simulink model "ParrotMinidroneKeyboardControl"  (R2025b)
settings: Solver=ode3  StartTime=0  StopTime=TFinal  FixedStep=Ts  RelTol=1e-3  EnableMultiTasking=on
values from neighbouring files (symbols this model uses):
  sensorCalibrationData = [0.09 -0.06 -9.473 -0.0095 -0.0075 0.0015 101270.95 0.2]    [sensorCalibration.mat]
undefined symbols (not defined in the file or in its folder): Command, ft, gcbh, init, m, Rec, s, SDTV, Sensors, States, stop_time, takeOffDuration, Ts, Vehicle, vrmfunc, VTs
libraries: simulink x16, aerolibconvert2 x4, SignalEditorBlockLib x2, environmentLibrary x2, visionconversions x2, visiongeotforms x2, aerolibutil x2, aerolibanimutils x1, aerolibnav x1, vrlib x1
(part 2 of 2)

== system ParrotMinidroneKeyboardControl/Simulink 3D Visualization/Simulink 3D/Euler to VR/Axis Angle Vector ==
  e0 : Inport
  2 : Gain  Gain=2  SaturateOnIntegerOverflow=on  OutDataTypeStr=Inherit: Same as input  ParamDataTypeStr=Inherit: Same as input
  Constant : Constant  Value=1e-6
  Demux : Demux  Outputs=[1 3 ]
      settings: DisplayOption=none
  Mux : Mux  Inputs=2
  Product : Product  Inputs=*/  InputSameDT=on  SaturateOnIntegerOverflow=on  OutDataTypeStr=Inherit: Same as first input
  Switch : Switch  Criteria=u2 ~= 0  SaturateOnIntegerOverflow=off  InputSameDT=off
  Trigonometric Function : Trigonometry
  Trigonometric Function2 : Trigonometry  Operator=acos
  e0_norm : Outport  VectorParamsAs1DForOutWhenUnconnected=off
  wires:
  Demux/1 -> Trigonometric Function2/1
  Demux/2 -> Product/1
  Mux/1 -> e0_norm/1
  Product/1 -> Mux/1
  2/1 -> Mux/2
  Trigonometric Function/1 -> Switch/1, Switch/2
  Trigonometric Function2/1 -> Trigonometric Function/1, 2/1
  e0/1 -> Demux/1
  Constant/1 -> Switch/3
  Switch/1 -> Product/2

== system ParrotMinidroneKeyboardControl/Simulink 3D Visualization/Simulink 3D/Euler to VR/Quaternion Normalization ==
  e0 : Inport
  1/2 : Gain  Gain=1/2  SaturateOnIntegerOverflow=on  OutDataTypeStr=Inherit: Same as input  ParamDataTypeStr=Inherit: Same as input
  Demux : Demux  Outputs=[1 3]
      settings: DisplayOption=none
  Mux : Mux  Inputs=2
  Product : Product  InputSameDT=on  SaturateOnIntegerOverflow=on  OutDataTypeStr=Inherit: Same as first input
  Trigonometric Function : Trigonometry
  Trigonometric Function1 : Trigonometry  Operator=cos
  e0_norm : Outport  VectorParamsAs1DForOutWhenUnconnected=off
  wires:
  Trigonometric Function1/1 -> Mux/1
  Demux/2 -> Product/2
  Demux/1 -> 1/2/1
  Mux/1 -> e0_norm/1
  Product/1 -> Mux/2
  Trigonometric Function/1 -> Product/1
  1/2/1 -> Trigonometric Function1/1, Trigonometric Function/1
  e0/1 -> Demux/1

== system ParrotMinidroneKeyboardControl/Simulink 3D Visualization/Simulink 3D/Euler to VR/Quaternion Normalization1 ==
  e0 : Inport
  1/2 : Gain  Gain=1/2  SaturateOnIntegerOverflow=on  OutDataTypeStr=Inherit: Same as input  ParamDataTypeStr=Inherit: Same as input
  Demux : Demux  Outputs=[1 3]
      settings: DisplayOption=none
  Mux : Mux  Inputs=2
  Product : Product  InputSameDT=on  SaturateOnIntegerOverflow=on  OutDataTypeStr=Inherit: Same as first input
  Trigonometric Function : Trigonometry
  Trigonometric Function1 : Trigonometry  Operator=cos
  e0_norm : Outport  VectorParamsAs1DForOutWhenUnconnected=off
  wires:
  e0/1 -> Demux/1
  1/2/1 -> Trigonometric Function/1, Trigonometric Function1/1
  Trigonometric Function/1 -> Product/1
  Product/1 -> Mux/2
  Mux/1 -> e0_norm/1
  Demux/1 -> 1/2/1
  Demux/2 -> Product/2
  Trigonometric Function1/1 -> Mux/1

== system ParrotMinidroneKeyboardControl/Simulink 3D Visualization/Simulink 3D/Euler to VR/Quaternion Normalization2 ==
  e0 : Inport
  1/2 : Gain  Gain=1/2  SaturateOnIntegerOverflow=on  OutDataTypeStr=Inherit: Same as input  ParamDataTypeStr=Inherit: Same as input
  Demux : Demux  Outputs=[1 3]
      settings: DisplayOption=none
  Mux : Mux  Inputs=2
  Product : Product  InputSameDT=on  SaturateOnIntegerOverflow=on  OutDataTypeStr=Inherit: Same as first input
  Trigonometric Function : Trigonometry
  Trigonometric Function1 : Trigonometry  Operator=cos
  e0_norm : Outport  VectorParamsAs1DForOutWhenUnconnected=off
  wires:
  Trigonometric Function1/1 -> Mux/1
  Demux/2 -> Product/2
  Demux/1 -> 1/2/1
  Mux/1 -> e0_norm/1
  Product/1 -> Mux/2
  Trigonometric Function/1 -> Product/1
  1/2/1 -> Trigonometric Function1/1, Trigonometric Function/1
  e0/1 -> Demux/1

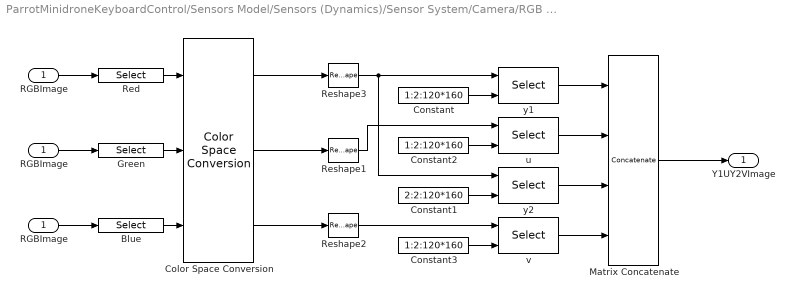
== system ParrotMinidroneKeyboardControl/Sensors Model/Sensors (Dynamics)/Sensor System/Camera/RGB to Y1UY2V1 ==
  RGBImage : Inport  OutDataTypeStr=uint8  PortDimensions=[120 160 3]
  " RGBImage " : InportShadow  OutDataTypeStr=uint8  PortDimensions=[120 160 3]
  Blue : Selector  NumberOfDimensions=3  InputPortWidth=3  IndexOptions=Select all,Select all,Index vector (dialog)  Indices=1,1,3  OutputSizes=1,1,1
  Color Space Conversion : visionconversions/Color Space  Conversion  conversion=Obsolete  conversionActive=R'G'B' to Y'CbCr  wp_str=D65  rec=Rec. 601 (SDTV)  sys=1125/60/2:1  imagePorts=Separate color signals
  Constant : Constant  Value=1:2:120*160
  Constant1 : Constant  Value=2:2:120*160
  Constant2 : Constant  Value=1:2:120*160
  Constant3 : Constant  Value=1:2:120*160
  Green : Selector  NumberOfDimensions=3  InputPortWidth=3  IndexOptions=Select all,Select all,Index vector (dialog)  Indices=1,1,2  OutputSizes=1,1,1
  Matrix Concatenate : Concatenate  NumInputs=4  Mode=Multidimensional array
  "RGBImage " : InportShadow  OutDataTypeStr=uint8  PortDimensions=[120 160 3]
  Red : Selector  NumberOfDimensions=3  InputPortWidth=3  IndexOptions=Select all,Select all,Index vector (dialog)  Indices=1,1,1  OutputSizes=1,1,1
  Reshape1 : Reshape  OutputDimensionality=Customize  OutputDimensions=[1,19200]
  Reshape2 : Reshape  OutputDimensionality=Customize  OutputDimensions=[1,19200]
  Reshape3 : Reshape  OutputDimensionality=Customize  OutputDimensions=[1,19200]
  u : Selector  InputPortWidth=120*160  IndexOptions=Index vector (port)  Indices=[1 3]  OutputSizes=1
  v : Selector  InputPortWidth=120*160  IndexOptions=Index vector (port)  Indices=[1 3]  OutputSizes=1
  y1 : Selector  InputPortWidth=120*160  IndexOptions=Index vector (port)  Indices=[1 3]  OutputSizes=1
  y2 : Selector  InputPortWidth=120*160  IndexOptions=Index vector (port)  Indices=[1 3]  OutputSizes=1
  Y1UY2VImage : Outport  OutDataTypeStr=uint8  PortDimensions=[4 9600]  VectorParamsAs1DForOutWhenUnconnected=off
  wires:
  v/1 -> Matrix Concatenate/4
  y1/1 -> Matrix Concatenate/1
  RGBImage/1 -> Green/1
  Red/1 -> Color Space Conversion/1
  Green/1 -> Color Space Conversion/2
  Blue/1 -> Color Space Conversion/3
  Reshape3/1 -> y1/1, y2/1
  Reshape1/1 -> u/1
  Reshape2/1 -> v/1
  Constant/1 -> y1/2
  Constant1/1 -> y2/2
  Constant2/1 -> u/2
  Constant3/1 -> v/2
  Matrix Concatenate/1 -> Y1UY2VImage/1
  u/1 -> Matrix Concatenate/2
  y2/1 -> Matrix Concatenate/3
  " RGBImage "/1 -> Red/1
  "RGBImage "/1 -> Blue/1
  Color Space Conversion/1 -> Reshape3/1
  Color Space Conversion/2 -> Reshape1/1
  Color Space Conversion/3 -> Reshape2/1

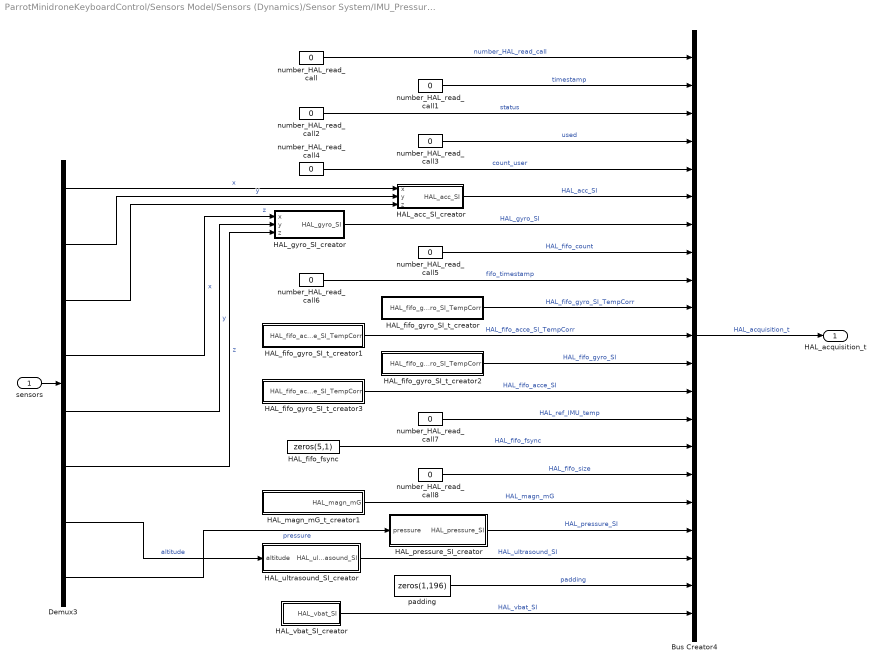
== system ParrotMinidroneKeyboardControl/Sensors Model/Sensors (Dynamics)/Sensor System/IMU_Pressure/HAL_acquisition_creator ==
  sensors : Inport
  Bus Creator4 : BusCreator  Inputs=21  OutDataTypeStr=Bus: HAL_acquisition_t  NonVirtualBus=on
      settings: InheritFromInputs=off
  Demux3 : Demux  Outputs=8
  HAL_acc_SI_creator : Subsystem
  HAL_fifo_fsync : Constant  Value=zeros(5,1)  OutDataTypeStr=uint8
  HAL_fifo_gyro_SI_t_creator : Subsystem
  HAL_fifo_gyro_SI_t_creator1 : Subsystem
  HAL_fifo_gyro_SI_t_creator2 : Subsystem
  HAL_fifo_gyro_SI_t_creator3 : Subsystem
  HAL_gyro_SI_creator : Subsystem
  HAL_magn_mG_t_creator1 : Subsystem
  HAL_pressure_SI_creator : Subsystem
  HAL_ultrasound_SI_creator : Subsystem
  HAL_vbat_SI_creator : Subsystem
  number_HAL_read_call : Constant  Value=0  OutDataTypeStr=int32
  number_HAL_read_call1 : Constant  Value=0  OutDataTypeStr=uint32
  number_HAL_read_call2 : Constant  Value=0  OutDataTypeStr=uint16
  number_HAL_read_call3 : Constant  Value=0  OutDataTypeStr=uint8
  number_HAL_read_call4 : Constant  Value=0  OutDataTypeStr=uint8
  number_HAL_read_call5 : Constant  Value=0  OutDataTypeStr=uint16
  number_HAL_read_call6 : Constant  Value=0  OutDataTypeStr=uint32
  number_HAL_read_call7 : Constant  Value=0  OutDataTypeStr=single
  number_HAL_read_call8 : Constant  Value=0  OutDataTypeStr=int32
  padding : Constant  Value=zeros(1,196)  OutDataTypeStr=uint8
  HAL_acquisition_t : Outport  OutDataTypeStr=Bus: HAL_acquisition_t  VectorParamsAs1DForOutWhenUnconnected=off
  wires:
  HAL_fifo_gyro_SI_t_creator1/1(HAL_fifo_acce_SI_TempCorr) -> Bus Creator4/11  "HAL_fifo_acce_SI_TempCorr"
  HAL_fifo_gyro_SI_t_creator2/1(HAL_fifo_gyro_SI_TempCorr) -> Bus Creator4/12  "HAL_fifo_gyro_SI"
  HAL_fifo_gyro_SI_t_creator3/1(HAL_fifo_acce_SI_TempCorr) -> Bus Creator4/13  "HAL_fifo_acce_SI"
  HAL_magn_mG_t_creator1/1(HAL_magn_mG) -> Bus Creator4/17  "HAL_magn_mG"
  HAL_fifo_fsync/1 -> Bus Creator4/15  "HAL_fifo_fsync"
  HAL_fifo_gyro_SI_t_creator/1(HAL_fifo_gyro_SI_TempCorr) -> Bus Creator4/10  "HAL_fifo_gyro_SI_TempCorr"
  number_HAL_read_call5/1 -> Bus Creator4/8  "HAL_fifo_count"
  number_HAL_read_call8/1 -> Bus Creator4/16  "HAL_fifo_size"
  number_HAL_read_call/1 -> Bus Creator4/1  "number_HAL_read_call"
  number_HAL_read_call2/1 -> Bus Creator4/3  "status"
  number_HAL_read_call3/1 -> Bus Creator4/4  "used"
  number_HAL_read_call6/1 -> Bus Creator4/9  "fifo_timestamp"
  number_HAL_read_call1/1 -> Bus Creator4/2  "timestamp"
  number_HAL_read_call4/1 -> Bus Creator4/5  "count_user"
  padding/1 -> Bus Creator4/20  "padding"
  number_HAL_read_call7/1 -> Bus Creator4/14  "HAL_ref_IMU_temp"
  HAL_vbat_SI_creator/1(HAL_vbat_SI) -> Bus Creator4/21  "HAL_vbat_SI"
  HAL_pressure_SI_creator/1(HAL_pressure_SI) -> Bus Creator4/18  "HAL_pressure_SI"
  Demux3/8 -> HAL_pressure_SI_creator/1(pressure)  "pressure"
  HAL_acc_SI_creator/1(HAL_acc_SI) -> Bus Creator4/6  "HAL_acc_SI"
  Demux3/3 -> HAL_acc_SI_creator/3(z)  "z"
  Demux3/2 -> HAL_acc_SI_creator/2(y)  "y"
  Demux3/1 -> HAL_acc_SI_creator/1(x)  "x"
  HAL_gyro_SI_creator/1(HAL_gyro_SI) -> Bus Creator4/7  "HAL_gyro_SI"
  Demux3/6 -> HAL_gyro_SI_creator/3(z)  "z"
  Demux3/5 -> HAL_gyro_SI_creator/2(y)  "y"
  Demux3/4 -> HAL_gyro_SI_creator/1(x)  "x"
  HAL_ultrasound_SI_creator/1(HAL_ultrasound_SI) -> Bus Creator4/19  "HAL_ultrasound_SI"
  Demux3/7 -> HAL_ultrasound_SI_creator/1(altitude)  "altitude"
  sensors/1 -> Demux3/1
  Bus Creator4/1 -> HAL_acquisition_t/1  "HAL_acquisition_t"

== system ParrotMinidroneKeyboardControl/Sensors Model/Sensors (Feedthrough)/Sensor System/Camera/RGB to Y1UY2V1 ==
  RGBImage : Inport  OutDataTypeStr=uint8  PortDimensions=[120 160 3]
  " RGBImage " : InportShadow  OutDataTypeStr=uint8  PortDimensions=[120 160 3]
  Blue : Selector  NumberOfDimensions=3  InputPortWidth=3  IndexOptions=Select all,Select all,Index vector (dialog)  Indices=1,1,3  OutputSizes=1,1,1
  Color Space Conversion : visionconversions/Color Space  Conversion  conversion=Obsolete  conversionActive=R'G'B' to Y'CbCr  wp_str=D65  rec=Rec. 601 (SDTV)  sys=1125/60/2:1  imagePorts=Separate color signals
  Constant : Constant  Value=1:2:120*160
  Constant1 : Constant  Value=2:2:120*160
  Constant2 : Constant  Value=1:2:120*160
  Constant3 : Constant  Value=1:2:120*160
  Green : Selector  NumberOfDimensions=3  InputPortWidth=3  IndexOptions=Select all,Select all,Index vector (dialog)  Indices=1,1,2  OutputSizes=1,1,1
  Matrix Concatenate : Concatenate  NumInputs=4  Mode=Multidimensional array
  "RGBImage " : InportShadow  OutDataTypeStr=uint8  PortDimensions=[120 160 3]
  Red : Selector  NumberOfDimensions=3  InputPortWidth=3  IndexOptions=Select all,Select all,Index vector (dialog)  Indices=1,1,1  OutputSizes=1,1,1
  Reshape1 : Reshape  OutputDimensionality=Customize  OutputDimensions=[1,19200]
  Reshape2 : Reshape  OutputDimensionality=Customize  OutputDimensions=[1,19200]
  Reshape3 : Reshape  OutputDimensionality=Customize  OutputDimensions=[1,19200]
  u : Selector  InputPortWidth=120*160  IndexOptions=Index vector (port)  Indices=[1 3]  OutputSizes=1
  v : Selector  InputPortWidth=120*160  IndexOptions=Index vector (port)  Indices=[1 3]  OutputSizes=1
  y1 : Selector  InputPortWidth=120*160  IndexOptions=Index vector (port)  Indices=[1 3]  OutputSizes=1
  y2 : Selector  InputPortWidth=120*160  IndexOptions=Index vector (port)  Indices=[1 3]  OutputSizes=1
  Y1UY2VImage : Outport  OutDataTypeStr=uint8  PortDimensions=[4 9600]  VectorParamsAs1DForOutWhenUnconnected=off
  wires:
  v/1 -> Matrix Concatenate/4
  y1/1 -> Matrix Concatenate/1
  RGBImage/1 -> Green/1
  Red/1 -> Color Space Conversion/1
  Green/1 -> Color Space Conversion/2
  Blue/1 -> Color Space Conversion/3
  Reshape3/1 -> y1/1, y2/1
  Reshape1/1 -> u/1
  Reshape2/1 -> v/1
  Constant/1 -> y1/2
  Constant1/1 -> y2/2
  Constant2/1 -> u/2
  Constant3/1 -> v/2
  Matrix Concatenate/1 -> Y1UY2VImage/1
  u/1 -> Matrix Concatenate/2
  y2/1 -> Matrix Concatenate/3
  " RGBImage "/1 -> Red/1
  "RGBImage "/1 -> Blue/1
  Color Space Conversion/1 -> Reshape3/1
  Color Space Conversion/2 -> Reshape1/1
  Color Space Conversion/3 -> Reshape2/1

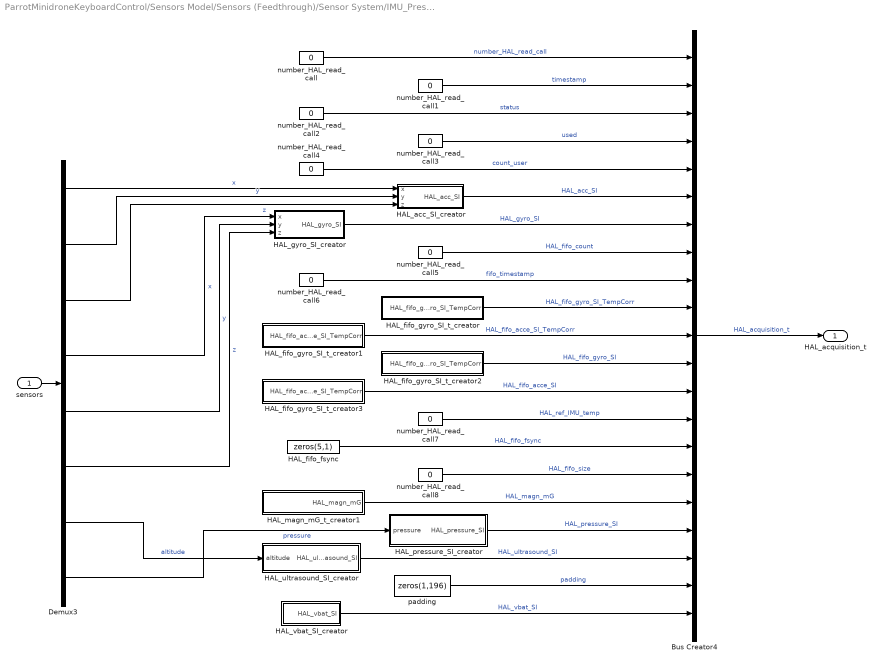
== system ParrotMinidroneKeyboardControl/Sensors Model/Sensors (Feedthrough)/Sensor System/IMU_Pressure/HAL_acquisition_creator ==
  sensors : Inport
  Bus Creator4 : BusCreator  Inputs=21  OutDataTypeStr=Bus: HAL_acquisition_t  NonVirtualBus=on
      settings: InheritFromInputs=off
  Demux3 : Demux  Outputs=8
  HAL_acc_SI_creator : Subsystem
  HAL_fifo_fsync : Constant  Value=zeros(5,1)  OutDataTypeStr=uint8
  HAL_fifo_gyro_SI_t_creator : Subsystem
  HAL_fifo_gyro_SI_t_creator1 : Subsystem
  HAL_fifo_gyro_SI_t_creator2 : Subsystem
  HAL_fifo_gyro_SI_t_creator3 : Subsystem
  HAL_gyro_SI_creator : Subsystem
  HAL_magn_mG_t_creator1 : Subsystem
  HAL_pressure_SI_creator : Subsystem
  HAL_ultrasound_SI_creator : Subsystem
  HAL_vbat_SI_creator : Subsystem
  number_HAL_read_call : Constant  Value=0  OutDataTypeStr=int32
  number_HAL_read_call1 : Constant  Value=0  OutDataTypeStr=uint32
  number_HAL_read_call2 : Constant  Value=0  OutDataTypeStr=uint16
  number_HAL_read_call3 : Constant  Value=0  OutDataTypeStr=uint8
  number_HAL_read_call4 : Constant  Value=0  OutDataTypeStr=uint8
  number_HAL_read_call5 : Constant  Value=0  OutDataTypeStr=uint16
  number_HAL_read_call6 : Constant  Value=0  OutDataTypeStr=uint32
  number_HAL_read_call7 : Constant  Value=0  OutDataTypeStr=single
  number_HAL_read_call8 : Constant  Value=0  OutDataTypeStr=int32
  padding : Constant  Value=zeros(1,196)  OutDataTypeStr=uint8
  HAL_acquisition_t : Outport  OutDataTypeStr=Bus: HAL_acquisition_t  VectorParamsAs1DForOutWhenUnconnected=off
  wires:
  HAL_fifo_gyro_SI_t_creator1/1(HAL_fifo_acce_SI_TempCorr) -> Bus Creator4/11  "HAL_fifo_acce_SI_TempCorr"
  HAL_fifo_gyro_SI_t_creator2/1(HAL_fifo_gyro_SI_TempCorr) -> Bus Creator4/12  "HAL_fifo_gyro_SI"
  HAL_fifo_gyro_SI_t_creator3/1(HAL_fifo_acce_SI_TempCorr) -> Bus Creator4/13  "HAL_fifo_acce_SI"
  HAL_magn_mG_t_creator1/1(HAL_magn_mG) -> Bus Creator4/17  "HAL_magn_mG"
  HAL_fifo_fsync/1 -> Bus Creator4/15  "HAL_fifo_fsync"
  HAL_fifo_gyro_SI_t_creator/1(HAL_fifo_gyro_SI_TempCorr) -> Bus Creator4/10  "HAL_fifo_gyro_SI_TempCorr"
  number_HAL_read_call5/1 -> Bus Creator4/8  "HAL_fifo_count"
  number_HAL_read_call8/1 -> Bus Creator4/16  "HAL_fifo_size"
  number_HAL_read_call/1 -> Bus Creator4/1  "number_HAL_read_call"
  number_HAL_read_call2/1 -> Bus Creator4/3  "status"
  number_HAL_read_call3/1 -> Bus Creator4/4  "used"
  number_HAL_read_call6/1 -> Bus Creator4/9  "fifo_timestamp"
  number_HAL_read_call1/1 -> Bus Creator4/2  "timestamp"
  number_HAL_read_call4/1 -> Bus Creator4/5  "count_user"
  padding/1 -> Bus Creator4/20  "padding"
  number_HAL_read_call7/1 -> Bus Creator4/14  "HAL_ref_IMU_temp"
  HAL_vbat_SI_creator/1(HAL_vbat_SI) -> Bus Creator4/21  "HAL_vbat_SI"
  HAL_pressure_SI_creator/1(HAL_pressure_SI) -> Bus Creator4/18  "HAL_pressure_SI"
  Demux3/8 -> HAL_pressure_SI_creator/1(pressure)  "pressure"
  HAL_acc_SI_creator/1(HAL_acc_SI) -> Bus Creator4/6  "HAL_acc_SI"
  Demux3/3 -> HAL_acc_SI_creator/3(z)  "z"
  Demux3/2 -> HAL_acc_SI_creator/2(y)  "y"
  Demux3/1 -> HAL_acc_SI_creator/1(x)  "x"
  HAL_gyro_SI_creator/1(HAL_gyro_SI) -> Bus Creator4/7  "HAL_gyro_SI"
  Demux3/6 -> HAL_gyro_SI_creator/3(z)  "z"
  Demux3/5 -> HAL_gyro_SI_creator/2(y)  "y"
  Demux3/4 -> HAL_gyro_SI_creator/1(x)  "x"
  HAL_ultrasound_SI_creator/1(HAL_ultrasound_SI) -> Bus Creator4/19  "HAL_ultrasound_SI"
  Demux3/7 -> HAL_ultrasound_SI_creator/1(altitude)  "altitude"
  sensors/1 -> Demux3/1
  Bus Creator4/1 -> HAL_acquisition_t/1  "HAL_acquisition_t"

== system ParrotMinidroneKeyboardControl/Sensors Model/Sensors (Dynamics)/Sensor System/IMU_Pressure/HAL_acquisition_creator/HAL_acc_SI_creator ==
  x : Inport
  y : Inport  Port=2
  z : Inport  Port=3
  Bus Creator : BusCreator  Inputs=4  OutDataTypeStr=Bus: HAL_acc_SI_t
  temperature : Constant  Value=0  OutDataTypeStr=single
  HAL_acc_SI : Outport  VectorParamsAs1DForOutWhenUnconnected=off
  wires:
  y/1 -> Bus Creator/2  "y"
  x/1 -> Bus Creator/1  "x"
  z/1 -> Bus Creator/3  "z"
  Bus Creator/1 -> HAL_acc_SI/1  "HAL_acc_SI"
  temperature/1 -> Bus Creator/4  "temperature"

== system ParrotMinidroneKeyboardControl/Sensors Model/Sensors (Dynamics)/Sensor System/IMU_Pressure/HAL_acquisition_creator/HAL_fifo_gyro_SI_t_creator ==
  Bus Creator : BusCreator  Inputs=3  OutDataTypeStr=Bus: HAL_fifo_gyro_SI_t  NonVirtualBus=on
      settings: InheritFromInputs=off
  Vector Concatenate : Concatenate  NumInputs=5
  z : Constant  Value=0  OutDataTypeStr=single
  z1 : Constant  Value=0  OutDataTypeStr=single
  z2 : Constant  Value=0  OutDataTypeStr=single
  HAL_fifo_gyro_SI_TempCorr : Outport  PortDimensions=5  VectorParamsAs1DForOutWhenUnconnected=off  LockScale=on
  wires:
  Vector Concatenate/1 -> HAL_fifo_gyro_SI_TempCorr/1
  Bus Creator/1 -> Vector Concatenate/3, Vector Concatenate/4, Vector Concatenate/5, Vector Concatenate/2, Vector Concatenate/1  "HAL_fifo_gyro_SI_TempCorr"
  z2/1 -> Bus Creator/1  "x"
  z/1 -> Bus Creator/3  "z"
  z1/1 -> Bus Creator/2  "y"

== system ParrotMinidroneKeyboardControl/Sensors Model/Sensors (Dynamics)/Sensor System/IMU_Pressure/HAL_acquisition_creator/HAL_fifo_gyro_SI_t_creator1 ==
  Bus Creator : BusCreator  Inputs=3  OutDataTypeStr=Bus: HAL_fifo_gyro_SI_t  NonVirtualBus=on
      settings: InheritFromInputs=off
  Vector Concatenate : Concatenate  NumInputs=5
  x : Constant  Value=0  OutDataTypeStr=single
  x1 : Constant  Value=0  OutDataTypeStr=single
  x2 : Constant  Value=0  OutDataTypeStr=single
  HAL_fifo_acce_SI_TempCorr : Outport  PortDimensions=5  VectorParamsAs1DForOutWhenUnconnected=off  LockScale=on
  wires:
  x1/1 -> Bus Creator/2  "y"
  x2/1 -> Bus Creator/3  "z"
  x/1 -> Bus Creator/1  "x"
  Bus Creator/1 -> Vector Concatenate/5, Vector Concatenate/4, Vector Concatenate/3, Vector Concatenate/2, Vector Concatenate/1  "HAL_fifo_gyro_SI_TempCorr"
  Vector Concatenate/1 -> HAL_fifo_acce_SI_TempCorr/1

== system ParrotMinidroneKeyboardControl/Sensors Model/Sensors (Dynamics)/Sensor System/IMU_Pressure/HAL_acquisition_creator/HAL_fifo_gyro_SI_t_creator2 ==
  Bus Creator : BusCreator  Inputs=3  OutDataTypeStr=Bus: HAL_fifo_gyro_SI_t  NonVirtualBus=on
      settings: InheritFromInputs=off
  Vector Concatenate : Concatenate  NumInputs=5
  z : Constant  Value=0  OutDataTypeStr=single
  z1 : Constant  Value=0  OutDataTypeStr=single
  z2 : Constant  Value=0  OutDataTypeStr=single
  HAL_fifo_gyro_SI_TempCorr : Outport  PortDimensions=5  VectorParamsAs1DForOutWhenUnconnected=off  LockScale=on
  wires:
  Vector Concatenate/1 -> HAL_fifo_gyro_SI_TempCorr/1
  Bus Creator/1 -> Vector Concatenate/3, Vector Concatenate/4, Vector Concatenate/5, Vector Concatenate/2, Vector Concatenate/1  "HAL_fifo_gyro_SI_TempCorr"
  z2/1 -> Bus Creator/1  "x"
  z/1 -> Bus Creator/3  "z"
  z1/1 -> Bus Creator/2  "y"

== system ParrotMinidroneKeyboardControl/Sensors Model/Sensors (Dynamics)/Sensor System/IMU_Pressure/HAL_acquisition_creator/HAL_fifo_gyro_SI_t_creator3 ==
  Bus Creator : BusCreator  Inputs=3  OutDataTypeStr=Bus: HAL_fifo_gyro_SI_t  NonVirtualBus=on
      settings: InheritFromInputs=off
  Vector Concatenate : Concatenate  NumInputs=5
  z : Constant  Value=0  OutDataTypeStr=single
  z1 : Constant  Value=0  OutDataTypeStr=single
  z2 : Constant  Value=0  OutDataTypeStr=single
  HAL_fifo_acce_SI_TempCorr : Outport  PortDimensions=5  VectorParamsAs1DForOutWhenUnconnected=off  LockScale=on
  wires:
  z1/1 -> Bus Creator/2  "y"
  z/1 -> Bus Creator/3  "z"
  z2/1 -> Bus Creator/1  "x"
  Bus Creator/1 -> Vector Concatenate/5, Vector Concatenate/4, Vector Concatenate/3, Vector Concatenate/2, Vector Concatenate/1  "HAL_fifo_gyro_SI_TempCorr"
  Vector Concatenate/1 -> HAL_fifo_acce_SI_TempCorr/1

== system ParrotMinidroneKeyboardControl/Sensors Model/Sensors (Dynamics)/Sensor System/IMU_Pressure/HAL_acquisition_creator/HAL_gyro_SI_creator ==
  x : Inport
  y : Inport  Port=2
  z : Inport  Port=3
  Bus Creator1 : BusCreator  Inputs=5  OutDataTypeStr=Bus: HAL_gyro_SI_t
  temperature : Constant  Value=0  OutDataTypeStr=single
  temperature_lsb : Constant  Value=0  OutDataTypeStr=int32
  HAL_gyro_SI : Outport  VectorParamsAs1DForOutWhenUnconnected=off
  wires:
  temperature/1 -> Bus Creator1/4  "temperature"
  z/1 -> Bus Creator1/3  "z"
  y/1 -> Bus Creator1/2  "y"
  x/1 -> Bus Creator1/1  "x"
  Bus Creator1/1 -> HAL_gyro_SI/1  "HAL_gyro_SI"
  temperature_lsb/1 -> Bus Creator1/5  "temperature_lsb"

== system ParrotMinidroneKeyboardControl/Sensors Model/Sensors (Dynamics)/Sensor System/IMU_Pressure/HAL_acquisition_creator/HAL_magn_mG_t_creator1 ==
  Bus Creator : BusCreator  Inputs=3  OutDataTypeStr=Bus: HAL_magn_mG_t
      settings: InheritFromInputs=off
  z : Constant  Value=0  OutDataTypeStr=single
  z1 : Constant  Value=0  OutDataTypeStr=single
  z2 : Constant  Value=0  OutDataTypeStr=single
  HAL_magn_mG : Outport  VectorParamsAs1DForOutWhenUnconnected=off
  wires:
  Bus Creator/1 -> HAL_magn_mG/1  "HAL_magn_mG"
  z1/1 -> Bus Creator/2  "y"
  z/1 -> Bus Creator/3  "z"
  z2/1 -> Bus Creator/1  "x"

== system ParrotMinidroneKeyboardControl/Sensors Model/Sensors (Dynamics)/Sensor System/IMU_Pressure/HAL_acquisition_creator/HAL_pressure_SI_creator ==
  pressure : Inport
  Bus Creator3 : BusCreator  Inputs=2  OutDataTypeStr=Bus: HAL_pressure_SI_t
  temperature : Constant  Value=0  OutDataTypeStr=double
  HAL_pressure_SI : Outport  VectorParamsAs1DForOutWhenUnconnected=off
  wires:
  pressure/1 -> Bus Creator3/2  "pressure"
  Bus Creator3/1 -> HAL_pressure_SI/1  "HAL_pressure_SI"
  temperature/1 -> Bus Creator3/1  "temperature"

== system ParrotMinidroneKeyboardControl/Sensors Model/Sensors (Dynamics)/Sensor System/IMU_Pressure/HAL_acquisition_creator/HAL_ultrasound_SI_creator ==
  altitude : Inport
  Bus Creator2 : BusCreator  Inputs=8  OutDataTypeStr=Bus: HAL_ultrasound_SI_t  NonVirtualBus=on
      settings: InheritFromInputs=off
  HAL_list_echo_t_creator : Subsystem
  HAL_list_echo_t_creator1 : Subsystem
  raw_altitude : Constant  Value=0  OutDataTypeStr=single
  raw_altitude1 : Constant  Value=0  OutDataTypeStr=uint16
  raw_altitude2 : Constant  Value=0  OutDataTypeStr=int32
  raw_altitude3 : Constant  Value=0  OutDataTypeStr=int32
  raw_altitude4 : Constant  Value=0  OutDataTypeStr=uint8
  HAL_ultrasound_SI : Outport  VectorParamsAs1DForOutWhenUnconnected=off
  wires:
  HAL_list_echo_t_creator1/1(HAL_list_echo) -> Bus Creator2/8  "HAL_list_echo_p"
  raw_altitude4/1 -> Bus Creator2/6  "new_data"
  raw_altitude/1 -> Bus Creator2/2  "raw_altitude"
  altitude/1 -> Bus Creator2/1  "altitude"
  Bus Creator2/1 -> HAL_ultrasound_SI/1  "HAL_ultrasound_SI"
  raw_altitude1/1 -> Bus Creator2/3  "nb_echo"
  raw_altitude2/1 -> Bus Creator2/4  "measure_ref"
  raw_altitude3/1 -> Bus Creator2/5  "measure_status"
  HAL_list_echo_t_creator/1(HAL_list_echo) -> Bus Creator2/7  "HAL_list_echo"

== system ParrotMinidroneKeyboardControl/Sensors Model/Sensors (Dynamics)/Sensor System/IMU_Pressure/HAL_acquisition_creator/HAL_vbat_SI_creator ==
  Bus Creator5 : BusCreator  Inputs=2  OutDataTypeStr=Bus: HAL_vbat_SI_t
  Demux4 : Demux  Outputs=2
  _DUMMY_batteryStatus : Constant  Value=Sensors.dummy.batteryStatus
  convert1 : DataTypeConversion  OutDataTypeStr=single  RndMeth=Floor
  convert2 : DataTypeConversion  OutDataTypeStr=uint32  RndMeth=Floor
  HAL_vbat_SI : Outport  VectorParamsAs1DForOutWhenUnconnected=off
  wires:
  Bus Creator5/1 -> HAL_vbat_SI/1  "HAL_vbat_SI"
  convert2/1 -> Bus Creator5/2  "vbat_percentage"
  convert1/1 -> Bus Creator5/1  "vbat_V"
  Demux4/2 -> convert2/1
  Demux4/1 -> convert1/1
  _DUMMY_batteryStatus/1 -> Demux4/1

== system ParrotMinidroneKeyboardControl/Sensors Model/Sensors (Feedthrough)/Sensor System/IMU_Pressure/HAL_acquisition_creator/HAL_acc_SI_creator ==
  x : Inport
  y : Inport  Port=2
  z : Inport  Port=3
  Bus Creator : BusCreator  Inputs=4  OutDataTypeStr=Bus: HAL_acc_SI_t
  temperature : Constant  Value=0  OutDataTypeStr=single
  HAL_acc_SI : Outport  VectorParamsAs1DForOutWhenUnconnected=off
  wires:
  y/1 -> Bus Creator/2  "y"
  x/1 -> Bus Creator/1  "x"
  z/1 -> Bus Creator/3  "z"
  Bus Creator/1 -> HAL_acc_SI/1  "HAL_acc_SI"
  temperature/1 -> Bus Creator/4  "temperature"

== system ParrotMinidroneKeyboardControl/Sensors Model/Sensors (Feedthrough)/Sensor System/IMU_Pressure/HAL_acquisition_creator/HAL_fifo_gyro_SI_t_creator ==
  Bus Creator : BusCreator  Inputs=3  OutDataTypeStr=Bus: HAL_fifo_gyro_SI_t  NonVirtualBus=on
      settings: InheritFromInputs=off
  Vector Concatenate : Concatenate  NumInputs=5
  z : Constant  Value=0  OutDataTypeStr=single
  z1 : Constant  Value=0  OutDataTypeStr=single
  z2 : Constant  Value=0  OutDataTypeStr=single
  HAL_fifo_gyro_SI_TempCorr : Outport  PortDimensions=5  VectorParamsAs1DForOutWhenUnconnected=off  LockScale=on
  wires:
  Vector Concatenate/1 -> HAL_fifo_gyro_SI_TempCorr/1
  Bus Creator/1 -> Vector Concatenate/3, Vector Concatenate/4, Vector Concatenate/5, Vector Concatenate/2, Vector Concatenate/1  "HAL_fifo_gyro_SI_TempCorr"
  z2/1 -> Bus Creator/1  "x"
  z/1 -> Bus Creator/3  "z"
  z1/1 -> Bus Creator/2  "y"

== system ParrotMinidroneKeyboardControl/Sensors Model/Sensors (Feedthrough)/Sensor System/IMU_Pressure/HAL_acquisition_creator/HAL_fifo_gyro_SI_t_creator1 ==
  Bus Creator : BusCreator  Inputs=3  OutDataTypeStr=Bus: HAL_fifo_gyro_SI_t  NonVirtualBus=on
      settings: InheritFromInputs=off
  Vector Concatenate : Concatenate  NumInputs=5
  x : Constant  Value=0  OutDataTypeStr=single
  x1 : Constant  Value=0  OutDataTypeStr=single
  x2 : Constant  Value=0  OutDataTypeStr=single
  HAL_fifo_acce_SI_TempCorr : Outport  PortDimensions=5  VectorParamsAs1DForOutWhenUnconnected=off  LockScale=on
  wires:
  x1/1 -> Bus Creator/2  "y"
  x2/1 -> Bus Creator/3  "z"
  x/1 -> Bus Creator/1  "x"
  Bus Creator/1 -> Vector Concatenate/5, Vector Concatenate/4, Vector Concatenate/3, Vector Concatenate/2, Vector Concatenate/1  "HAL_fifo_gyro_SI_TempCorr"
  Vector Concatenate/1 -> HAL_fifo_acce_SI_TempCorr/1

== system ParrotMinidroneKeyboardControl/Sensors Model/Sensors (Feedthrough)/Sensor System/IMU_Pressure/HAL_acquisition_creator/HAL_fifo_gyro_SI_t_creator2 ==
  Bus Creator : BusCreator  Inputs=3  OutDataTypeStr=Bus: HAL_fifo_gyro_SI_t  NonVirtualBus=on
      settings: InheritFromInputs=off
  Vector Concatenate : Concatenate  NumInputs=5
  z : Constant  Value=0  OutDataTypeStr=single
  z1 : Constant  Value=0  OutDataTypeStr=single
  z2 : Constant  Value=0  OutDataTypeStr=single
  HAL_fifo_gyro_SI_TempCorr : Outport  PortDimensions=5  VectorParamsAs1DForOutWhenUnconnected=off  LockScale=on
  wires:
  Vector Concatenate/1 -> HAL_fifo_gyro_SI_TempCorr/1
  Bus Creator/1 -> Vector Concatenate/3, Vector Concatenate/4, Vector Concatenate/5, Vector Concatenate/2, Vector Concatenate/1  "HAL_fifo_gyro_SI_TempCorr"
  z2/1 -> Bus Creator/1  "x"
  z/1 -> Bus Creator/3  "z"
  z1/1 -> Bus Creator/2  "y"

== system ParrotMinidroneKeyboardControl/Sensors Model/Sensors (Feedthrough)/Sensor System/IMU_Pressure/HAL_acquisition_creator/HAL_fifo_gyro_SI_t_creator3 ==
  Bus Creator : BusCreator  Inputs=3  OutDataTypeStr=Bus: HAL_fifo_gyro_SI_t  NonVirtualBus=on
      settings: InheritFromInputs=off
  Vector Concatenate : Concatenate  NumInputs=5
  z : Constant  Value=0  OutDataTypeStr=single
  z1 : Constant  Value=0  OutDataTypeStr=single
  z2 : Constant  Value=0  OutDataTypeStr=single
  HAL_fifo_acce_SI_TempCorr : Outport  PortDimensions=5  VectorParamsAs1DForOutWhenUnconnected=off  LockScale=on
  wires:
  z1/1 -> Bus Creator/2  "y"
  z/1 -> Bus Creator/3  "z"
  z2/1 -> Bus Creator/1  "x"
  Bus Creator/1 -> Vector Concatenate/5, Vector Concatenate/4, Vector Concatenate/3, Vector Concatenate/2, Vector Concatenate/1  "HAL_fifo_gyro_SI_TempCorr"
  Vector Concatenate/1 -> HAL_fifo_acce_SI_TempCorr/1

== system ParrotMinidroneKeyboardControl/Sensors Model/Sensors (Feedthrough)/Sensor System/IMU_Pressure/HAL_acquisition_creator/HAL_gyro_SI_creator ==
  x : Inport
  y : Inport  Port=2
  z : Inport  Port=3
  Bus Creator1 : BusCreator  Inputs=5  OutDataTypeStr=Bus: HAL_gyro_SI_t
  temperature : Constant  Value=0  OutDataTypeStr=single
  temperature_lsb : Constant  Value=0  OutDataTypeStr=int32
  HAL_gyro_SI : Outport  VectorParamsAs1DForOutWhenUnconnected=off
  wires:
  temperature/1 -> Bus Creator1/4  "temperature"
  z/1 -> Bus Creator1/3  "z"
  y/1 -> Bus Creator1/2  "y"
  x/1 -> Bus Creator1/1  "x"
  Bus Creator1/1 -> HAL_gyro_SI/1  "HAL_gyro_SI"
  temperature_lsb/1 -> Bus Creator1/5  "temperature_lsb"

== system ParrotMinidroneKeyboardControl/Sensors Model/Sensors (Feedthrough)/Sensor System/IMU_Pressure/HAL_acquisition_creator/HAL_magn_mG_t_creator1 ==
  Bus Creator : BusCreator  Inputs=3  OutDataTypeStr=Bus: HAL_magn_mG_t
      settings: InheritFromInputs=off
  z : Constant  Value=0  OutDataTypeStr=single
  z1 : Constant  Value=0  OutDataTypeStr=single
  z2 : Constant  Value=0  OutDataTypeStr=single
  HAL_magn_mG : Outport  VectorParamsAs1DForOutWhenUnconnected=off
  wires:
  Bus Creator/1 -> HAL_magn_mG/1  "HAL_magn_mG"
  z1/1 -> Bus Creator/2  "y"
  z/1 -> Bus Creator/3  "z"
  z2/1 -> Bus Creator/1  "x"

== system ParrotMinidroneKeyboardControl/Sensors Model/Sensors (Feedthrough)/Sensor System/IMU_Pressure/HAL_acquisition_creator/HAL_pressure_SI_creator ==
  pressure : Inport
  Bus Creator3 : BusCreator  Inputs=2  OutDataTypeStr=Bus: HAL_pressure_SI_t
  temperature : Constant  Value=0  OutDataTypeStr=double
  HAL_pressure_SI : Outport  VectorParamsAs1DForOutWhenUnconnected=off
  wires:
  pressure/1 -> Bus Creator3/2  "pressure"
  Bus Creator3/1 -> HAL_pressure_SI/1  "HAL_pressure_SI"
  temperature/1 -> Bus Creator3/1  "temperature"

== system ParrotMinidroneKeyboardControl/Sensors Model/Sensors (Feedthrough)/Sensor System/IMU_Pressure/HAL_acquisition_creator/HAL_ultrasound_SI_creator ==
  altitude : Inport
  Bus Creator2 : BusCreator  Inputs=8  OutDataTypeStr=Bus: HAL_ultrasound_SI_t  NonVirtualBus=on
      settings: InheritFromInputs=off
  HAL_list_echo_t_creator : Subsystem
  HAL_list_echo_t_creator1 : Subsystem
  raw_altitude : Constant  Value=0  OutDataTypeStr=single
  raw_altitude1 : Constant  Value=0  OutDataTypeStr=uint16
  raw_altitude2 : Constant  Value=0  OutDataTypeStr=int32
  raw_altitude3 : Constant  Value=0  OutDataTypeStr=int32
  raw_altitude4 : Constant  Value=0  OutDataTypeStr=uint8
  HAL_ultrasound_SI : Outport  VectorParamsAs1DForOutWhenUnconnected=off
  wires:
  HAL_list_echo_t_creator1/1(HAL_list_echo) -> Bus Creator2/8  "HAL_list_echo_p"
  raw_altitude4/1 -> Bus Creator2/6  "new_data"
  raw_altitude/1 -> Bus Creator2/2  "raw_altitude"
  altitude/1 -> Bus Creator2/1  "altitude"
  Bus Creator2/1 -> HAL_ultrasound_SI/1  "HAL_ultrasound_SI"
  raw_altitude1/1 -> Bus Creator2/3  "nb_echo"
  raw_altitude2/1 -> Bus Creator2/4  "measure_ref"
  raw_altitude3/1 -> Bus Creator2/5  "measure_status"
  HAL_list_echo_t_creator/1(HAL_list_echo) -> Bus Creator2/7  "HAL_list_echo"

== system ParrotMinidroneKeyboardControl/Sensors Model/Sensors (Feedthrough)/Sensor System/IMU_Pressure/HAL_acquisition_creator/HAL_vbat_SI_creator ==
  Bus Creator5 : BusCreator  Inputs=2  OutDataTypeStr=Bus: HAL_vbat_SI_t
  Demux4 : Demux  Outputs=2
  _DUMMY_batteryStatus : Constant  Value=Sensors.dummy.batteryStatus
  convert1 : DataTypeConversion  OutDataTypeStr=single  RndMeth=Floor
  convert2 : DataTypeConversion  OutDataTypeStr=uint32  RndMeth=Floor
  HAL_vbat_SI : Outport  VectorParamsAs1DForOutWhenUnconnected=off
  wires:
  Bus Creator5/1 -> HAL_vbat_SI/1  "HAL_vbat_SI"
  convert2/1 -> Bus Creator5/2  "vbat_percentage"
  convert1/1 -> Bus Creator5/1  "vbat_V"
  Demux4/2 -> convert2/1
  Demux4/1 -> convert1/1
  _DUMMY_batteryStatus/1 -> Demux4/1

== system ParrotMinidroneKeyboardControl/Sensors Model/Sensors (Dynamics)/Sensor System/IMU_Pressure/HAL_acquisition_creator/HAL_ultrasound_SI_creator/HAL_list_echo_t_creator ==
  Bus Creator7 : BusCreator  Inputs=2  OutDataTypeStr=Bus: HAL_list_echo_t  NonVirtualBus=on
  HAL_echo_t_creator : Subsystem
  Vector Concatenate : Concatenate  NumInputs=30
  number_of_echoes : Constant  Value=0  OutDataTypeStr=uint8
  HAL_list_echo : Outport  VectorParamsAs1DForOutWhenUnconnected=off
  wires:
  HAL_echo_t_creator/1(HAL_echo_t) -> Vector Concatenate/1, Vector Concatenate/2, Vector Concatenate/3, Vector Concatenate/4, Vector Concatenate/5, Vector Concatenate/6, Vector Concatenate/7, Vector Concatenate/8, Vector Concatenate/9, Vector Concatenate/10, Vector Concatenate/11, Vector Concatenate/12, Vector Concatenate/13, Vector Concatenate/14, Vector Concatenate/15, Vector Concatenate/16, Vector Concatenate/17, Vector Concatenate/18, Vector Concatenate/19, Vector Concatenate/20, Vector Concatenate/21, Vector Concatenate/22, Vector Concatenate/23, Vector Concatenate/24, Vector Concatenate/25, Vector Concatenate/26, Vector Concatenate/27, Vector Concatenate/28, Vector Concatenate/29, Vector Concatenate/30
  Vector Concatenate/1 -> Bus Creator7/1  "tab_echo"
  Bus Creator7/1 -> HAL_list_echo/1  "HAL_list_echo"
  number_of_echoes/1 -> Bus Creator7/2  "number_of_echoes"

== system ParrotMinidroneKeyboardControl/Sensors Model/Sensors (Dynamics)/Sensor System/IMU_Pressure/HAL_acquisition_creator/HAL_ultrasound_SI_creator/HAL_list_echo_t_creator1 ==
  Bus Creator7 : BusCreator  Inputs=2  OutDataTypeStr=Bus: HAL_list_echo_t  NonVirtualBus=on
  HAL_echo_t_creator : Subsystem
  Vector Concatenate : Concatenate  NumInputs=30
  number_of_echoes : Constant  Value=0  OutDataTypeStr=uint8
  HAL_list_echo : Outport  VectorParamsAs1DForOutWhenUnconnected=off
  wires:
  number_of_echoes/1 -> Bus Creator7/2  "number_of_echoes"
  Bus Creator7/1 -> HAL_list_echo/1  "HAL_list_echo"
  Vector Concatenate/1 -> Bus Creator7/1  "tab_echo"
  HAL_echo_t_creator/1(HAL_echo_t) -> Vector Concatenate/30, Vector Concatenate/29, Vector Concatenate/28, Vector Concatenate/27, Vector Concatenate/26, Vector Concatenate/25, Vector Concatenate/24, Vector Concatenate/23, Vector Concatenate/22, Vector Concatenate/21, Vector Concatenate/20, Vector Concatenate/19, Vector Concatenate/18, Vector Concatenate/17, Vector Concatenate/16, Vector Concatenate/15, Vector Concatenate/14, Vector Concatenate/13, Vector Concatenate/12, Vector Concatenate/11, Vector Concatenate/10, Vector Concatenate/9, Vector Concatenate/8, Vector Concatenate/7, Vector Concatenate/6, Vector Concatenate/5, Vector Concatenate/4, Vector Concatenate/3, Vector Concatenate/2, Vector Concatenate/1

== system ParrotMinidroneKeyboardControl/Sensors Model/Sensors (Feedthrough)/Sensor System/IMU_Pressure/HAL_acquisition_creator/HAL_ultrasound_SI_creator/HAL_list_echo_t_creator ==
  Bus Creator7 : BusCreator  Inputs=2  OutDataTypeStr=Bus: HAL_list_echo_t  NonVirtualBus=on
  HAL_echo_t_creator : Subsystem
  Vector Concatenate : Concatenate  NumInputs=30
  number_of_echoes : Constant  Value=0  OutDataTypeStr=uint8
  HAL_list_echo : Outport  VectorParamsAs1DForOutWhenUnconnected=off
  wires:
  HAL_echo_t_creator/1(HAL_echo_t) -> Vector Concatenate/1, Vector Concatenate/2, Vector Concatenate/3, Vector Concatenate/4, Vector Concatenate/5, Vector Concatenate/6, Vector Concatenate/7, Vector Concatenate/8, Vector Concatenate/9, Vector Concatenate/10, Vector Concatenate/11, Vector Concatenate/12, Vector Concatenate/13, Vector Concatenate/14, Vector Concatenate/15, Vector Concatenate/16, Vector Concatenate/17, Vector Concatenate/18, Vector Concatenate/19, Vector Concatenate/20, Vector Concatenate/21, Vector Concatenate/22, Vector Concatenate/23, Vector Concatenate/24, Vector Concatenate/25, Vector Concatenate/26, Vector Concatenate/27, Vector Concatenate/28, Vector Concatenate/29, Vector Concatenate/30
  Vector Concatenate/1 -> Bus Creator7/1  "tab_echo"
  Bus Creator7/1 -> HAL_list_echo/1  "HAL_list_echo"
  number_of_echoes/1 -> Bus Creator7/2  "number_of_echoes"

== system ParrotMinidroneKeyboardControl/Sensors Model/Sensors (Feedthrough)/Sensor System/IMU_Pressure/HAL_acquisition_creator/HAL_ultrasound_SI_creator/HAL_list_echo_t_creator1 ==
  Bus Creator7 : BusCreator  Inputs=2  OutDataTypeStr=Bus: HAL_list_echo_t  NonVirtualBus=on
  HAL_echo_t_creator : Subsystem
  Vector Concatenate : Concatenate  NumInputs=30
  number_of_echoes : Constant  Value=0  OutDataTypeStr=uint8
  HAL_list_echo : Outport  VectorParamsAs1DForOutWhenUnconnected=off
  wires:
  number_of_echoes/1 -> Bus Creator7/2  "number_of_echoes"
  Bus Creator7/1 -> HAL_list_echo/1  "HAL_list_echo"
  Vector Concatenate/1 -> Bus Creator7/1  "tab_echo"
  HAL_echo_t_creator/1(HAL_echo_t) -> Vector Concatenate/30, Vector Concatenate/29, Vector Concatenate/28, Vector Concatenate/27, Vector Concatenate/26, Vector Concatenate/25, Vector Concatenate/24, Vector Concatenate/23, Vector Concatenate/22, Vector Concatenate/21, Vector Concatenate/20, Vector Concatenate/19, Vector Concatenate/18, Vector Concatenate/17, Vector Concatenate/16, Vector Concatenate/15, Vector Concatenate/14, Vector Concatenate/13, Vector Concatenate/12, Vector Concatenate/11, Vector Concatenate/10, Vector Concatenate/9, Vector Concatenate/8, Vector Concatenate/7, Vector Concatenate/6, Vector Concatenate/5, Vector Concatenate/4, Vector Concatenate/3, Vector Concatenate/2, Vector Concatenate/1

== system ParrotMinidroneKeyboardControl/Sensors Model/Sensors (Dynamics)/Sensor System/IMU_Pressure/HAL_acquisition_creator/HAL_ultrasound_SI_creator/HAL_list_echo_t_creator/HAL_echo_t_creator ==
  Bus Creator6 : BusCreator  Inputs=7  OutDataTypeStr=Bus: HAL_echo_t  NonVirtualBus=on
  begin_echo_index{,1,4,6} (4 alike) : Constant  Value=0  OutDataTypeStr=uint16
  begin_echo_index2 : Constant  Value=0  OutDataTypeStr=int16
  begin_echo_index3 : Constant  Value=0  OutDataTypeStr=int32
  begin_echo_index5 : Constant  Value=0  OutDataTypeStr=int16
  HAL_echo_t : Outport  OutDataTypeStr=Bus: HAL_echo_t  VectorParamsAs1DForOutWhenUnconnected=off
  wires:
  begin_echo_index6/1 -> Bus Creator6/7  "pre_max_index"
  begin_echo_index5/1 -> Bus Creator6/6  "d_echo"
  begin_echo_index4/1 -> Bus Creator6/5  "precedent"
  begin_echo_index3/1 -> Bus Creator6/4  "max_value"
  begin_echo_index2/1 -> Bus Creator6/3  "max_value_index"
  begin_echo_index1/1 -> Bus Creator6/2  "end_echo_index"
  begin_echo_index/1 -> Bus Creator6/1  "begin_echo_index"
  Bus Creator6/1 -> HAL_echo_t/1  "HAL_echo_t"

== system ParrotMinidroneKeyboardControl/Sensors Model/Sensors (Dynamics)/Sensor System/IMU_Pressure/HAL_acquisition_creator/HAL_ultrasound_SI_creator/HAL_list_echo_t_creator1/HAL_echo_t_creator ==
  Bus Creator6 : BusCreator  Inputs=7  OutDataTypeStr=Bus: HAL_echo_t  NonVirtualBus=on
  begin_echo_index{,1,4,6} (4 alike) : Constant  Value=0  OutDataTypeStr=uint16
  begin_echo_index2 : Constant  Value=0  OutDataTypeStr=int16
  begin_echo_index3 : Constant  Value=0  OutDataTypeStr=int32
  begin_echo_index5 : Constant  Value=0  OutDataTypeStr=int16
  HAL_echo_t : Outport  OutDataTypeStr=Bus: HAL_echo_t  VectorParamsAs1DForOutWhenUnconnected=off
  wires:
  Bus Creator6/1 -> HAL_echo_t/1  "HAL_echo_t"
  begin_echo_index/1 -> Bus Creator6/1  "begin_echo_index"
  begin_echo_index1/1 -> Bus Creator6/2  "end_echo_index"
  begin_echo_index2/1 -> Bus Creator6/3  "max_value_index"
  begin_echo_index3/1 -> Bus Creator6/4  "max_value"
  begin_echo_index4/1 -> Bus Creator6/5  "precedent"
  begin_echo_index5/1 -> Bus Creator6/6  "d_echo"
  begin_echo_index6/1 -> Bus Creator6/7  "pre_max_index"

== system ParrotMinidroneKeyboardControl/Sensors Model/Sensors (Feedthrough)/Sensor System/IMU_Pressure/HAL_acquisition_creator/HAL_ultrasound_SI_creator/HAL_list_echo_t_creator/HAL_echo_t_creator ==
  Bus Creator6 : BusCreator  Inputs=7  OutDataTypeStr=Bus: HAL_echo_t  NonVirtualBus=on
  begin_echo_index{,1,4,6} (4 alike) : Constant  Value=0  OutDataTypeStr=uint16
  begin_echo_index2 : Constant  Value=0  OutDataTypeStr=int16
  begin_echo_index3 : Constant  Value=0  OutDataTypeStr=int32
  begin_echo_index5 : Constant  Value=0  OutDataTypeStr=int16
  HAL_echo_t : Outport  OutDataTypeStr=Bus: HAL_echo_t  VectorParamsAs1DForOutWhenUnconnected=off
  wires:
  begin_echo_index6/1 -> Bus Creator6/7  "pre_max_index"
  begin_echo_index5/1 -> Bus Creator6/6  "d_echo"
  begin_echo_index4/1 -> Bus Creator6/5  "precedent"
  begin_echo_index3/1 -> Bus Creator6/4  "max_value"
  begin_echo_index2/1 -> Bus Creator6/3  "max_value_index"
  begin_echo_index1/1 -> Bus Creator6/2  "end_echo_index"
  begin_echo_index/1 -> Bus Creator6/1  "begin_echo_index"
  Bus Creator6/1 -> HAL_echo_t/1  "HAL_echo_t"

== system ParrotMinidroneKeyboardControl/Sensors Model/Sensors (Feedthrough)/Sensor System/IMU_Pressure/HAL_acquisition_creator/HAL_ultrasound_SI_creator/HAL_list_echo_t_creator1/HAL_echo_t_creator ==
  Bus Creator6 : BusCreator  Inputs=7  OutDataTypeStr=Bus: HAL_echo_t  NonVirtualBus=on
  begin_echo_index{,1,4,6} (4 alike) : Constant  Value=0  OutDataTypeStr=uint16
  begin_echo_index2 : Constant  Value=0  OutDataTypeStr=int16
  begin_echo_index3 : Constant  Value=0  OutDataTypeStr=int32
  begin_echo_index5 : Constant  Value=0  OutDataTypeStr=int16
  HAL_echo_t : Outport  OutDataTypeStr=Bus: HAL_echo_t  VectorParamsAs1DForOutWhenUnconnected=off
  wires:
  Bus Creator6/1 -> HAL_echo_t/1  "HAL_echo_t"
  begin_echo_index/1 -> Bus Creator6/1  "begin_echo_index"
  begin_echo_index1/1 -> Bus Creator6/2  "end_echo_index"
  begin_echo_index2/1 -> Bus Creator6/3  "max_value_index"
  begin_echo_index3/1 -> Bus Creator6/4  "max_value"
  begin_echo_index4/1 -> Bus Creator6/5  "precedent"
  begin_echo_index5/1 -> Bus Creator6/6  "d_echo"
  begin_echo_index6/1 -> Bus Creator6/7  "pre_max_index"
